simulink model "InvertedPendulum_Plant"  (R2023a)
settings: Solver=ode4  StartTime=0.0  StopTime=5  FixedStep=0.001  RelTol=1e-3
settings Model: Creator=Fasih  LastModifiedBy=Fasih

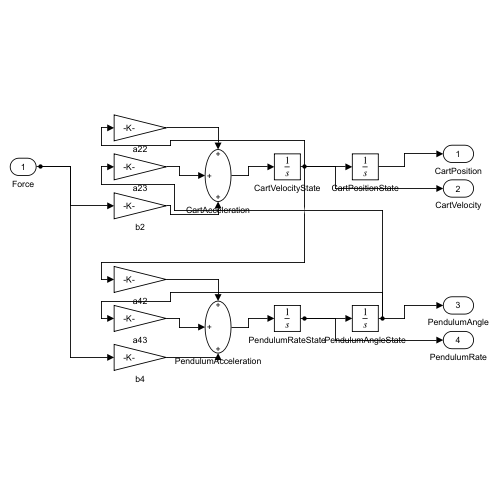
[thumbnail: Simulink's stored preview of the top-level diagram]
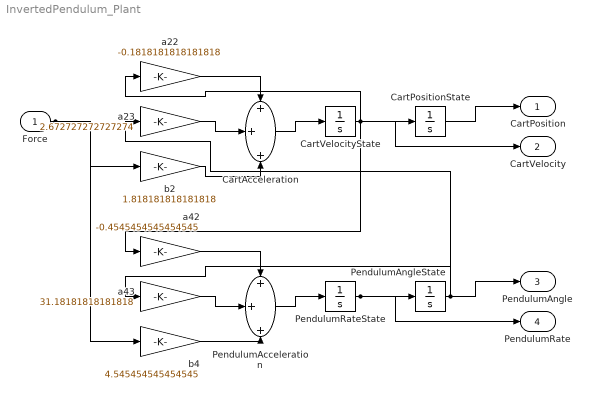
== system InvertedPendulum_Plant ==
  Force : Inport
  CartAcceleration : Sum  Inputs=+++
  CartPositionState : Integrator
  CartVelocityState : Integrator
  PendulumAcceleration : Sum  Inputs=+++
  PendulumAngleState : Integrator  InitialCondition=0.08
  PendulumRateState : Integrator
  a22 : Gain  Gain=-0.1818181818181818
  a23 : Gain  Gain=2.672727272727274
  a42 : Gain  Gain=-0.4545454545454545
  a43 : Gain  Gain=31.18181818181818
  b2 : Gain  Gain=1.818181818181818
  b4 : Gain  Gain=4.545454545454545
  CartPosition : Outport
  CartVelocity : Outport  Port=2
  PendulumAngle : Outport  Port=3
  PendulumRate : Outport  Port=4
  wires:
  CartVelocityState/1 -> a22/1, CartPositionState/1, a42/1, CartVelocity/1
  PendulumAngleState/1 -> a23/1, a43/1, PendulumAngle/1
  Force/1 -> b2/1, b4/1
  a22/1 -> CartAcceleration/1
  a23/1 -> CartAcceleration/2
  b2/1 -> CartAcceleration/3
  CartAcceleration/1 -> CartVelocityState/1
  a42/1 -> PendulumAcceleration/1
  a43/1 -> PendulumAcceleration/2
  b4/1 -> PendulumAcceleration/3
  PendulumAcceleration/1 -> PendulumRateState/1
  PendulumRateState/1 -> PendulumAngleState/1, PendulumRate/1
  CartPositionState/1 -> CartPosition/1
